simulink model "simpleFuselage_lib_example"  (R2018b)
settings: Solver=FixedStepAuto  StartTime=0.0  StopTime=100  FixedStep=0.01  RelTol=1e-3
libraries: simpleFuselage_lib x1
settings Model: Creator=Yannic  LastModifiedBy=fabian

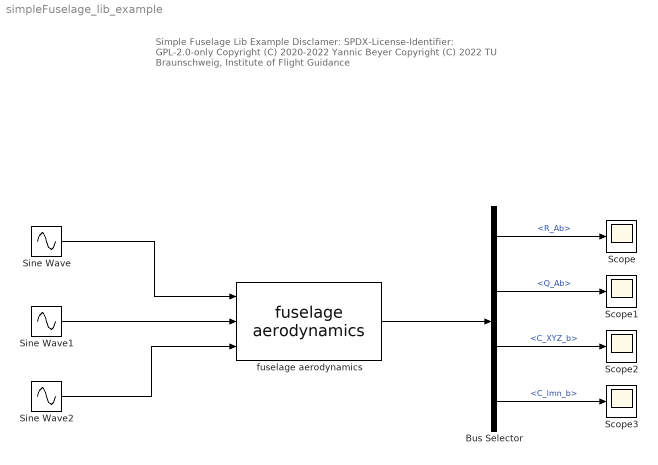
== system simpleFuselage_lib_example ==
  note: Simple Fuselage Lib Example
      |
      | Disclamer:
      | SPDX-License-Identifier: GPL-2.0-only
      |
      | Copyright (C) 2020-2022 Yannic Beyer
      | Copyright (C) 2022 TU Braunschweig, Institute of Flight Guidance
  Bus Selector : BusSelector  OutputSignals=R_Ab,Q_Ab,C_XYZ_b,C_lmn_b
  Scope{,1..3} (4 alike) : Scope
  Sine Wave : Sin  Amplitude=0.1  Frequency=0.2  SampleTime=0
  Sine Wave1 : Sin  Amplitude=0.1  Bias=10  Frequency=0.1  SampleTime=0
  Sine Wave2 : Sin  Amplitude=10  Bias=1000  Frequency=0.08  SampleTime=0
  fuselage aerodynamics : simpleFuselage_lib/fuselage aerodynamics  simple_fuselage=simple_fuselage
  wires:
  Sine Wave/1 -> fuselage aerodynamics/1
  Sine Wave1/1 -> fuselage aerodynamics/2
  Sine Wave2/1 -> fuselage aerodynamics/3
  fuselage aerodynamics/1 -> Bus Selector/1
  Bus Selector/1 -> Scope/1  "<R_Ab>"
  Bus Selector/2 -> Scope1/1  "<Q_Ab>"
  Bus Selector/3 -> Scope2/1  "<C_XYZ_b>"
  Bus Selector/4 -> Scope3/1  "<C_lmn_b>"
